simulink model "mos"  (R2024a)
settings: Solver=VariableStepAuto  StartTime=0.0  StopTime=0.06  RelTol=1e-3
libraries: spsDCVoltageSourceLib x1, spsMosfetLib x1, spsSeriesRLCBranchLib x1, spsVoltageMeasurementLib x1, sps_lib x1
settings Model: Creator=Adithyan  LastModifiedBy=Adithyan

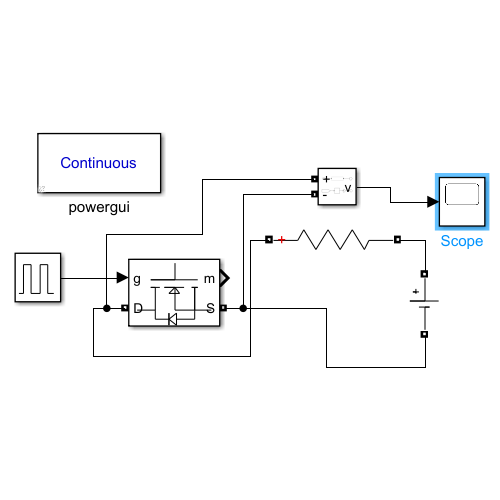
[thumbnail: Simulink's stored preview of the top-level diagram]
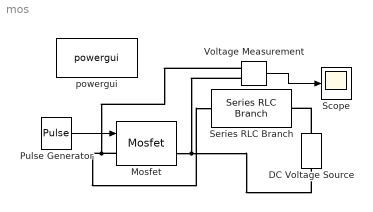
== system mos ==
  DC Voltage Source : spsDCVoltageSourceLib/DC Voltage Source  Amplitude=12  Measurements=None
  Mosfet : spsMosfetLib/Mosfet  Ron=0.1  Lon=0  Rd=0.01  Vfd=0  IC=0  Rs=1e5  Cs=inf  Measurements=on
  Pulse Generator : DiscretePulseGenerator  PulseType=Time based  Amplitude=10  Period=10  PulseWidth=5
  Scope : Scope
  Series RLC Branch : spsSeriesRLCBranchLib/Series RLC Branch  LConnTagsString=__new0  RConnTagsString=__new0  BranchType=R  Resistance=100  Inductance=1e-3  SetiL0=off  InitialCurrent=0  Capacitance=1e-6  Setx0=off  InitialVoltage=0  Measurements=None
  Voltage Measurement : spsVoltageMeasurementLib/Voltage Measurement  PhasorSimulation=off  OutputType=Complex  PSBequivalent=0
  powergui : sps_lib/powergui  Priority=1  SimulationMode=Continuous  SampleTime=50e-6  frequency=60  Iterations=50  frequencyindice=0  Pbase=100e6  ErrMax=1e-4  UnitsV=kV  UnitsW=MW  buscounter=0  FunctionMessages=off  echomessages=off  EnableUseOfTLC=off  CurrentSourceSwitches=off  DisableSnubberDevices=off  DisableRonSwitches=off  DisableVfSwitches=off  DisplayEquations=off  AutomaticDiscreteSolvers=off  SolverType=Tustin/Backward Euler (TBE)  Interpol=off  ExternalGateDelay=off  methode=off  Ts=100  x0status=blocks  SPID=on  SwTol=0  HookPort=off  NonlinearTolerance=1e-4  nMaxIteration=100  ContinueOnMaxIteration=off  RestoreLinks=warning  ResistiveCurrentMeasurement=off  Frange=[0:2:500]  Ylog=off  Xlog=on  ShowGrid=off  save=off  variable=ZData  structure=0  ZoomFFT=off  StartTime=0.0  cycles=1  DisplayStyle=1  fundamental=60  FreqAxis=off  MaxFrequency=1000  frequencyindicesteady=1  RmsSteady=1  display=off
  wires:
  Pulse Generator/1 -> Mosfet/1
  Voltage Measurement/1 -> Scope/1
  connections:
  DC Voltage Source/RConn1 -- Series RLC Branch/RConn1
  Mosfet/LConn1 -- Voltage Measurement/LConn1 -- Series RLC Branch/LConn1
  Mosfet/RConn1 -- Voltage Measurement/LConn2 -- DC Voltage Source/LConn1
